simulink model "controlw6DOFfreedomandFlightGear"  (R2026b)
settings: Solver=ode4  StopTime=120  FixedStep=0.005
values from neighbouring files (symbols this model uses):
  g = 9.81    [NatFreq_Calcs.m]    (also in QuadrotorEOM.m = params.g; QuadrotorPlant.m = params.g; eigCheckTemp.m; init_quadrotor.m)
  Kdphi = Kd_mult / J_inv(1,1)    [NatFreq_Calcs.m]    (also in eigCheckTemp.m = 0.92686; init_quadrotor.m = 0.53463)
  Kdpsi = (2 * zeta_yaw * wn_yaw) / J_inv(3,3)    [NatFreq_Calcs.m]    (also in eigCheckTemp.m = 0.05506; init_quadrotor.m = 0.69126)
  Kdtheta = Kd_mult / J_inv(2,2)    [NatFreq_Calcs.m]    (also in eigCheckTemp.m = 0.55207; init_quadrotor.m = 0.90628)
  Kdz = (2 * zeta_z * wn_z) * m    [NatFreq_Calcs.m]    (also in eigCheckTemp.m = 6.13958; init_quadrotor.m = 12.28992)
  Kiphi = Kpphi * 0.05    [NatFreq_Calcs.m]    (also in eigCheckTemp.m = 2.44895; init_quadrotor.m = 0.70645)
  Kipsi = Kppsi * 0.05    [NatFreq_Calcs.m]    (also in eigCheckTemp.m = 0.01652; init_quadrotor.m = 0.68766)
  Kitheta = Kptheta * 0.05    [NatFreq_Calcs.m]    (also in eigCheckTemp.m = 1.4587; init_quadrotor.m = 1.19753)
  Kiz = 0.0    (= 0)    [NatFreq_Calcs.m]    (also in eigCheckTemp.m = 1.08057; init_quadrotor.m)
  Kpphi = Kp_mult / J_inv(1,1)    [NatFreq_Calcs.m]    (also in eigCheckTemp.m = 24.48955; init_quadrotor.m = 14.12894)
  Kppsi = (wn_yaw^2) / J_inv(3,3)    [NatFreq_Calcs.m]    (also in eigCheckTemp.m = 0.16519; init_quadrotor.m = 13.75321)
  Kptheta = Kp_mult / J_inv(2,2)    [NatFreq_Calcs.m]    (also in eigCheckTemp.m = 14.58697; init_quadrotor.m = 23.95062)
  Kpu = (2 * zeta_mid * wn_mid) / g    [NatFreq_Calcs.m]    (also in eigCheckTemp.m = 0.81125; init_quadrotor.m = 3.245)
  Kpv = Kpu    [NatFreq_Calcs.m]    (also in eigCheckTemp.m = 0.81125; init_quadrotor.m = 3.245)
  Kpx = wn_outer    [NatFreq_Calcs.m]    (also in eigCheckTemp.m = 0.39792; init_quadrotor.m = 1.59167)
  Kpy = Kpx    [NatFreq_Calcs.m]    (also in eigCheckTemp.m = 0.39792; init_quadrotor.m = 1.59167)
  Kpz = (wn_z^2) * m    [NatFreq_Calcs.m]    (also in eigCheckTemp.m = 10.80567; init_quadrotor.m = 24.45186)
  m = 1544.28/1000    (= 1.54428)    [NatFreq_Calcs.m]    (also in PlotAircraftSim.m = 256; QuadrotorEOM.m = params.m; QuadrotorPlant.m = params.m; eigCheckTemp.m = 0.8721)
undefined symbols (not defined in the file or in its folder): dragCoeffVec, rho
libraries: aerolibfltsims x2, aerolibanimutils x1
settings Model: SimulationMode=accelerator  Creator=YoYo  LastModifiedBy=YoYo
settings SolverCC: MinimalZcImpactIntegration=on
settings DataIOCC: DSMLogging=off  ReturnWorkspaceOutputs=off  SaveOutput=off  SaveTime=off
settings DebuggingCC: MultiTaskDSMMsg=none  ReadBeforeWriteMsg=DisableAll  WriteAfterReadMsg=DisableAll  WriteAfterWriteMsg=DisableAll
settings SFSimCC: SFSimEcho=off

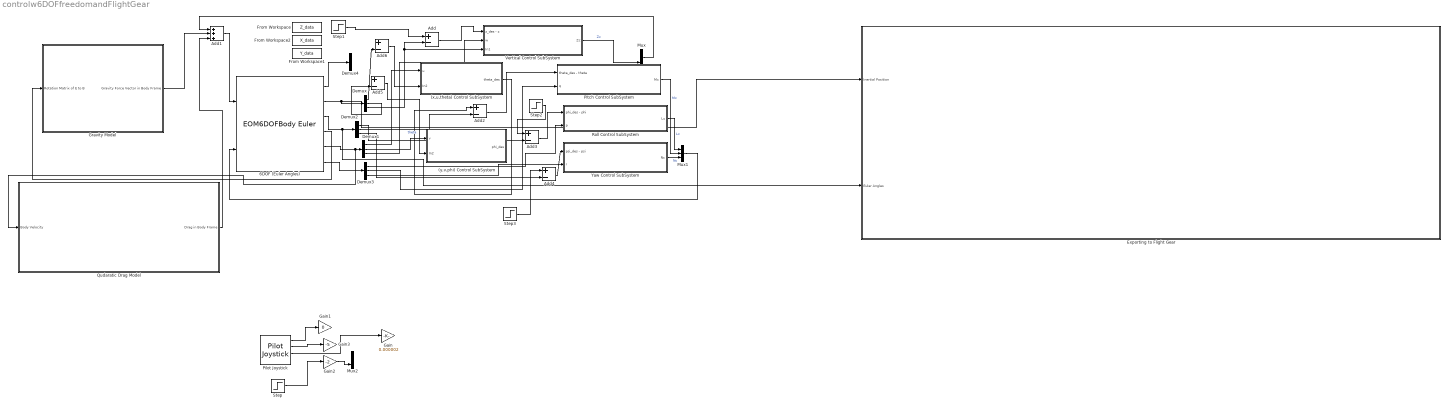
== system controlw6DOFfreedomandFlightGear ==
  (x,u,theta) Control SubSystem : Subsystem
  (y,v,phi) Control SubSystem : Subsystem
  6DOF (Euler Angles) : EOM6DOFBodyEuler  mass_0=m  inertia=I
  Add{,2..6} (6 alike) : Sum  Inputs=+-
  Add1 : Sum  Inputs=+++
  Demux{,1..4} (5 alike) : Demux  Outputs=3
  Exporting to Flight Gear : Subsystem
  From Workspace : FromWorkspace  VariableName=Z_data
  From Workspace1 : FromWorkspace  VariableName=Y_data
  From Workspace2 : FromWorkspace  VariableName=X_data
  Gain : Gain  Gain=0.000002
  Gain1 : Gain  Gain=0
  Gain2 : Gain  Gain=-2
  Gain3 : Gain  Gain=-5
  Gravity Model : Subsystem
  Mux : Mux  Inputs=3
  Mux1 : Mux  Inputs=3
  Mux2 : Mux  Inputs=3
  Pilot Joystick : aerolibanimutils/Pilot Joystick  JoystickID=None  OutputConfiguration=FourAxis  SampleTime=0.02  action=Error
  Pitch Control SubSystem : Subsystem
  Qudaratic Drag Model : Subsystem
  Roll Control SubSystem : Subsystem
  Step : Step  SampleTime=3
  Step1 : Step  Time=2  FinalValue=-2  SampleTime=0
  Step2 : Step  Time=2  FinalValue=0  SampleTime=0
  Step3 : Step  Time=2  FinalValue=0  SampleTime=0
  Vertical Control SubSystem : Subsystem
  Yaw Control SubSystem : Subsystem
  wires:
  6DOF (Euler Angles)/2 -> Exporting to Flight Gear/1(Inertial Position), Demux/1
  Demux/3 -> Add/2, Vertical Control SubSystem/3(In1)
  Add/1 -> Vertical Control SubSystem/1(z_des - z)
  6DOF (Euler Angles)/5 -> Qudaratic Drag Model/1(Body Velocity), Demux1/1
  Demux1/3 -> Vertical Control SubSystem/2(w)
  Vertical Control SubSystem/1(Zc) -> Mux/3  "Zc"
  Add1/1 -> 6DOF (Euler Angles)/1
  6DOF (Euler Angles)/4 -> Gravity Model/1(Rotation Matrix of E to B)
  Gravity Model/1(Gravity Force Vector in Body Frame) -> Add1/2
  Qudaratic Drag Model/1(Drag in Body Frame) -> Add1/3
  6DOF (Euler Angles)/3 -> Exporting to Flight Gear/2(Euler Angles), Demux2/1
  Demux2/2 -> Add2/2  "theta"
  Add2/1 -> Pitch Control SubSystem/1(theta_des - theta)
  6DOF (Euler Angles)/6 -> Demux3/1
  Demux3/2 -> Pitch Control SubSystem/2(q)
  Pitch Control SubSystem/1(Mc) -> Mux1/2  "Mc"
  Mux1/1 -> 6DOF (Euler Angles)/2
  Demux3/1 -> Roll Control SubSystem/2(p)
  Gain2/1 -> Mux2/3
  Pilot Joystick/2 -> Gain3/1
  Demux2/1 -> Add3/2
  Pilot Joystick/1 -> Gain1/1
  Add3/1 -> Roll Control SubSystem/1(phi_des - phi)
  Roll Control SubSystem/1(Lc) -> Mux1/1  "Lc"
  Mux/1 -> Add1/1
  Add4/1 -> Yaw Control SubSystem/1(psi_des - psi)
  Demux2/3 -> Add4/2
  Demux3/3 -> Yaw Control SubSystem/2(r)
  Pilot Joystick/3 -> Gain/1
  6DOF (Euler Angles)/1 -> Demux4/1
  Step/1 -> Gain2/1
  Demux1/1 -> (x,u,theta) Control SubSystem/1(u)
  (x,u,theta) Control SubSystem/1(theta_des) -> Add2/1
  Add6/1 -> (x,u,theta) Control SubSystem/2(In2)
  Demux/1 -> Add6/2
  Demux1/2 -> (y,v,phi) Control SubSystem/1(v)
  Demux/2 -> Add5/2
  Add5/1 -> (y,v,phi) Control SubSystem/2(In2)
  Step3/1 -> Add4/1
  Step1/1 -> Add/1
  Step2/1 -> Add3/1
  Yaw Control SubSystem/1(Nc) -> Mux1/3  "Nc"

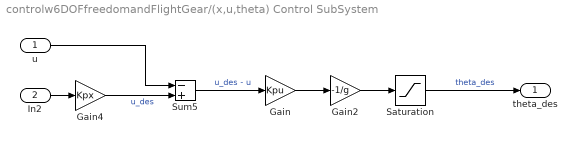
== system controlw6DOFfreedomandFlightGear/(x,u,theta) Control SubSystem ==
  u : Inport
  In2 : Inport  Port=2
  Gain : Gain  Gain=Kpu
  Gain2 : Gain  Gain=-1/g
  Gain4 : Gain  Gain=Kpx
  Saturation : Saturate  UpperLimit=0.25  LowerLimit=-0.25
  Sum5 : Sum  Inputs=-+
  theta_des : Outport
  wires:
  Sum5/1 -> Gain/1  "u_des - u"
  u/1 -> Sum5/1
  Gain4/1 -> Sum5/2  "u_des"
  In2/1 -> Gain4/1
  Saturation/1 -> theta_des/1  "theta_des"
  Gain/1 -> Gain2/1
  Gain2/1 -> Saturation/1

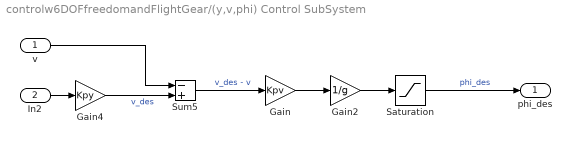
== system controlw6DOFfreedomandFlightGear/(y,v,phi) Control SubSystem ==
  v : Inport
  In2 : Inport  Port=2
  Gain : Gain  Gain=Kpv
  Gain2 : Gain  Gain=1/g
  Gain4 : Gain  Gain=Kpy
  Saturation : Saturate  UpperLimit=0.25  LowerLimit=-0.25
  Sum5 : Sum  Inputs=-+
  phi_des : Outport
  wires:
  Sum5/1 -> Gain/1  "v_des - v"
  v/1 -> Sum5/1
  Gain4/1 -> Sum5/2  "v_des"
  In2/1 -> Gain4/1
  Saturation/1 -> phi_des/1  "phi_des"
  Gain/1 -> Gain2/1
  Gain2/1 -> Saturation/1

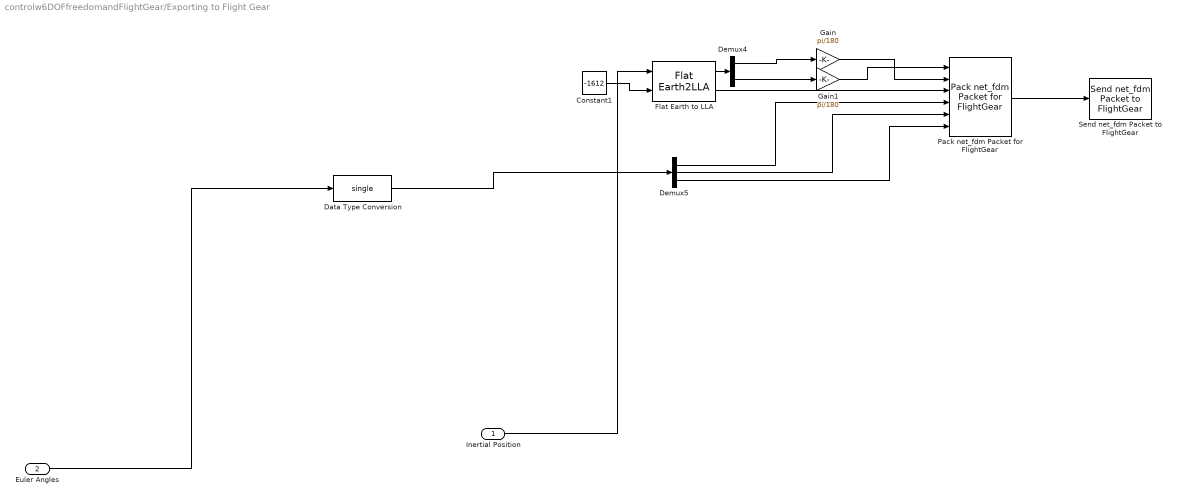
== system controlw6DOFfreedomandFlightGear/Exporting to Flight Gear ==
  Inertial Position : Inport
  Euler Angles : Inport  Port=2
  Constant1 : Constant  Value=-1612
  Data Type Conversion : DataTypeConversion  OutDataTypeStr=single  SaturateOnIntegerOverflow=off  RndMeth=Floor
  Demux4 : Demux  Outputs=2
  Demux5 : Demux  Outputs=3
  Flat Earth to LLA : FlatEarth2LLA  LL0=[40.039365 -105.226090]
  Gain : Gain  Gain=pi/180
  Gain1 : Gain  Gain=pi/180
  Pack net_fdm Packet for FlightGear : aerolibfltsims/Pack net_fdm Packet for FlightGear  FlightGearVersion=v2019.1  ShowPositionAttitudeInputs=on  ShowVelocityAccelerationInputs=off  ShowControlSurfacePositionInputs=off  ShowEngineFuelInputs=off  ShowLandingGearInputs=off  ShowEnvironmentInputs=off  SampleTime=0.01  packetVersion=24
  Send net_fdm Packet to FlightGear : aerolibfltsims/Send net_fdm Packet to FlightGear  DestinationIpAddress=127.0.0.1  DestinationPort=5503  LocalIpPort=-1  varLen=off  SampleTime=0.01
  wires:
  Demux4/1 -> Gain/1
  Demux5/3 -> Pack net_fdm Packet for FlightGear/6
  Pack net_fdm Packet for FlightGear/1 -> Send net_fdm Packet to FlightGear/1
  Gain/1 -> Pack net_fdm Packet for FlightGear/2
  Flat Earth to LLA/1 -> Demux4/1
  Demux4/2 -> Gain1/1
  Gain1/1 -> Pack net_fdm Packet for FlightGear/1
  Constant1/1 -> Flat Earth to LLA/2
  Flat Earth to LLA/2 -> Pack net_fdm Packet for FlightGear/3
  Demux5/1 -> Pack net_fdm Packet for FlightGear/4
  Demux5/2 -> Pack net_fdm Packet for FlightGear/5
  Data Type Conversion/1 -> Demux5/1
  Inertial Position/1 -> Flat Earth to LLA/1
  Euler Angles/1 -> Data Type Conversion/1

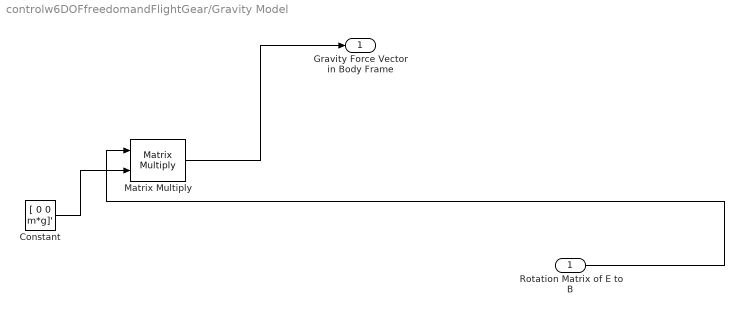
== system controlw6DOFfreedomandFlightGear/Gravity Model ==
  Rotation Matrix of E to B : Inport
  Constant : Constant  Value=[ 0 0 m*g]'
  Matrix Multiply : Product  Multiplication=Matrix(*)
  Gravity Force Vector in Body Frame : Outport
  wires:
  Constant/1 -> Matrix Multiply/2
  Matrix Multiply/1 -> Gravity Force Vector in Body Frame/1
  Rotation Matrix of E to B/1 -> Matrix Multiply/1

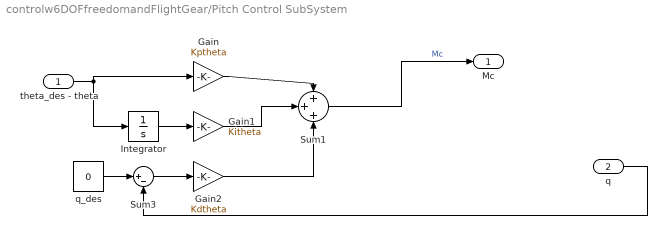
== system controlw6DOFfreedomandFlightGear/Pitch Control SubSystem ==
  theta_des - theta : Inport
  q : Inport  Port=2
  Gain : Gain  Gain=Kptheta
  Gain1 : Gain  Gain=Kitheta
  Gain2 : Gain  Gain=Kdtheta
  Integrator : Integrator  LimitOutput=on  UpperSaturationLimit=500  LowerSaturationLimit=-500
  Sum1 : Sum  Inputs=+++
  Sum3 : Sum  Inputs=|+-
  q_des : Constant  Value=0
  Mc : Outport
  wires:
  Sum1/1 -> Mc/1  "Mc"
  theta_des - theta/1 -> Integrator/1, Gain/1
  q/1 -> Sum3/2
  Gain/1 -> Sum1/1
  Sum3/1 -> Gain2/1
  Integrator/1 -> Gain1/1
  q_des/1 -> Sum3/1
  Gain1/1 -> Sum1/2
  Gain2/1 -> Sum1/3

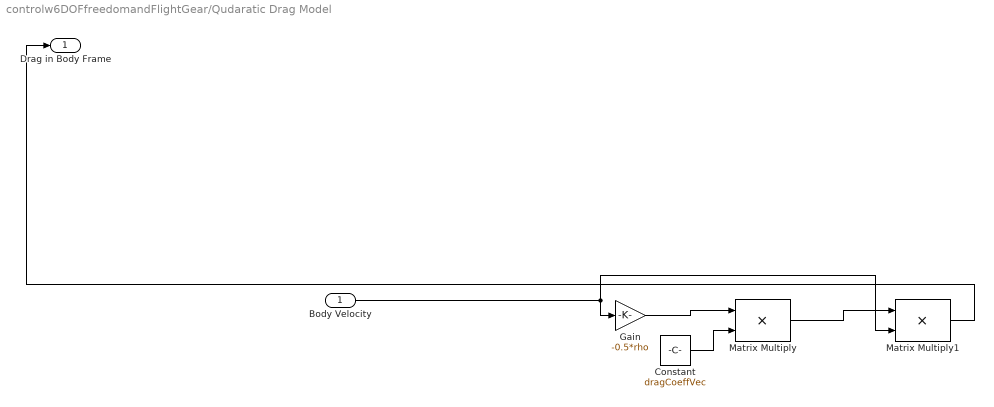
== system controlw6DOFfreedomandFlightGear/Qudaratic Drag Model ==
  Body Velocity : Inport
  Constant : Constant  Value=dragCoeffVec
  Gain : Gain  Gain=-0.5*rho
  Matrix Multiply : Product
  Matrix Multiply1 : Product
  Drag in Body Frame : Outport
  wires:
  Matrix Multiply/1 -> Matrix Multiply1/1
  Gain/1 -> Matrix Multiply/1
  Body Velocity/1 -> Gain/1, Matrix Multiply1/2
  Constant/1 -> Matrix Multiply/2
  Matrix Multiply1/1 -> Drag in Body Frame/1

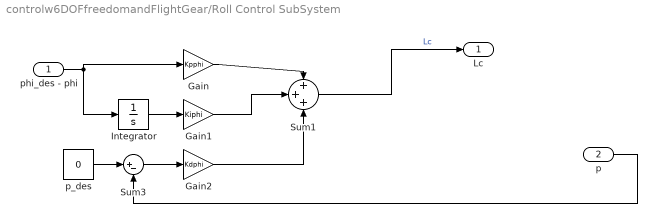
== system controlw6DOFfreedomandFlightGear/Roll Control SubSystem ==
  phi_des - phi : Inport
  p : Inport  Port=2
  Gain : Gain  Gain=Kpphi
  Gain1 : Gain  Gain=Kiphi
  Gain2 : Gain  Gain=Kdphi
  Integrator : Integrator  LimitOutput=on  UpperSaturationLimit=500  LowerSaturationLimit=-500
  Sum1 : Sum  Inputs=+++
  Sum3 : Sum  Inputs=|+-
  p_des : Constant  Value=0
  Lc : Outport
  wires:
  Sum1/1 -> Lc/1  "Lc"
  phi_des - phi/1 -> Integrator/1, Gain/1
  p/1 -> Sum3/2
  Gain/1 -> Sum1/1
  Sum3/1 -> Gain2/1
  Integrator/1 -> Gain1/1
  Gain1/1 -> Sum1/2
  Gain2/1 -> Sum1/3
  p_des/1 -> Sum3/1

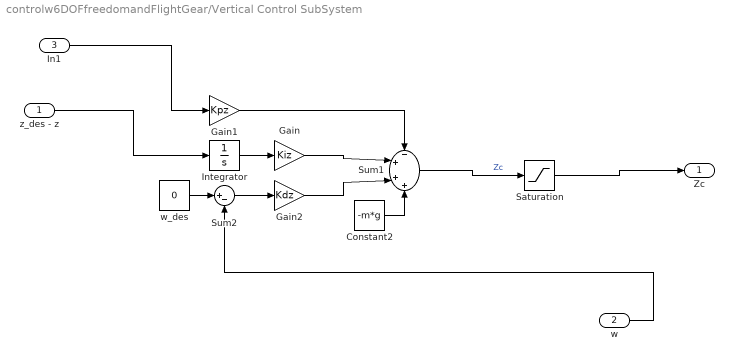
== system controlw6DOFfreedomandFlightGear/Vertical Control SubSystem ==
  z_des - z : Inport
  w : Inport  Port=2
  In1 : Inport  Port=3
  Constant2 : Constant  Value=-m*g
  Gain : Gain  Gain=Kiz
  Gain1 : Gain  Gain=Kpz
  Gain2 : Gain  Gain=Kdz
  Integrator : Integrator  LimitOutput=on  UpperSaturationLimit=500  LowerSaturationLimit=-500
  Saturation : Saturate  UpperLimit=0  LowerLimit=-300
  Sum1 : Sum  Inputs=-+++
  Sum2 : Sum  Inputs=|+-
  w_des : Constant  Value=0
  Zc : Outport
  wires:
  w/1 -> Sum2/2
  Constant2/1 -> Sum1/4
  Gain1/1 -> Sum1/1
  w_des/1 -> Sum2/1
  Integrator/1 -> Gain/1
  Sum2/1 -> Gain2/1
  Gain2/1 -> Sum1/3
  Gain/1 -> Sum1/2
  Sum1/1 -> Saturation/1  "Zc"
  Saturation/1 -> Zc/1
  z_des - z/1 -> Integrator/1
  In1/1 -> Gain1/1

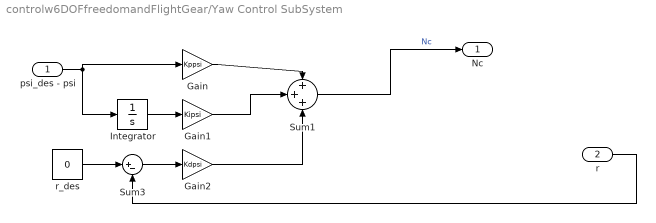
== system controlw6DOFfreedomandFlightGear/Yaw Control SubSystem ==
  psi_des - psi : Inport
  r : Inport  Port=2
  Gain : Gain  Gain=Kppsi
  Gain1 : Gain  Gain=Kipsi
  Gain2 : Gain  Gain=Kdpsi
  Integrator : Integrator  LimitOutput=on  UpperSaturationLimit=500  LowerSaturationLimit=-500
  Sum1 : Sum  Inputs=+++
  Sum3 : Sum  Inputs=|+-
  r_des : Constant  Value=0
  Nc : Outport
  wires:
  Sum1/1 -> Nc/1  "Nc"
  psi_des - psi/1 -> Integrator/1, Gain/1
  r/1 -> Sum3/2
  Sum3/1 -> Gain2/1
  Integrator/1 -> Gain1/1
  r_des/1 -> Sum3/1
  Gain2/1 -> Sum1/3
  Gain/1 -> Sum1/1
  Gain1/1 -> Sum1/2
